simulink model "tb_structure"  (R2026b)
model workspace (MAT data in the model file):
  tbs.t = [0 1000000]
  tbs.uL = [0 0]
  tbs.uR = [0 0]
  tbs.rref = [0 0]
  tbs.pi_on = 0
  tbs.pi_Kp = 0.4
  tbs.pi_Ki = 2
  tbs.pi_lim = 0.4
  tbs.kw = 4.63333333333
  tbs.t_impl = [0 1000000]
  tbs.w_impl = [0 0]
  tbs.nozzleOn = [0; 0; 0; 0; 0; 0; 0; 0]
  tbs.liftDuty = 0
  tbs.envdist.F_ext_B = [0; 0; 0]
  tbs.envdist.M_ext_B = [0; 0; 0]
  tbs.envovr.use_T = 0
  tbs.envovr.T_amb = 318.15
  tbs.envovr.use_G = 0
  tbs.envovr.G_solar = 0
  tbs.envovr.use_soil = 0
  tbs.envovr.soil_id = 2
  tbs.envovr.dock_contact_force = 0
  tbs.decim = 10
undefined symbols (not defined in the file or in its folder): DiscIntNeverNeededParam, Ts
libraries: fl_lib x8, nesl_utility x7
settings Model: Creator=aomar  LastModifiedBy=aomar

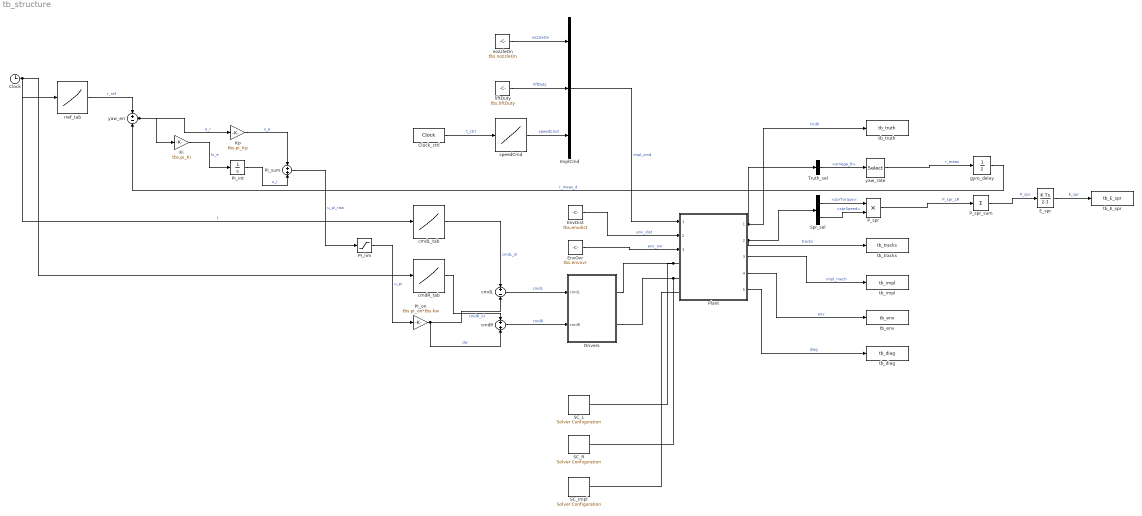
== system tb_structure ==
  Clock : Clock
  Clock_ctrl : DigitalClock  SampleTime=Ts.ctrl
  Drivers : Subsystem  Variant=on  VariantControlMode=label  LabelModeActiveChoice=speed
  E_spr : DiscreteIntegrator  gainval=1  SampleTime=Ts.base  ICPrevOutput=DiscIntNeverNeededParam  ICPrevScaledInput=DiscIntNeverNeededParam
  EnvDist : Constant  Value=tbs.envdist  OutDataTypeStr=Bus: Bus_EnvDisturbance  SampleTime=Ts.base
  EnvOvr : Constant  Value=tbs.envovr  OutDataTypeStr=Bus: Bus_EnvOverride  SampleTime=Ts.env
  ImplCmd : BusCreator  Inputs=3  OutDataTypeStr=Bus: Bus_ImplementCmd  NonVirtualBus=on
  Ki : Gain  Gain=tbs.pi_Ki
  Kp : Gain  Gain=tbs.pi_Kp
  PI_int : Integrator  LimitOutput=on  UpperSaturationLimit=tbs.pi_lim  LowerSaturationLimit=-tbs.pi_lim
  PI_lim : Saturate  UpperLimit=tbs.pi_lim  LowerLimit=-tbs.pi_lim
  PI_on : Gain  Gain=tbs.pi_on*tbs.kw
  PI_sum : Sum
  P_spr : Product  Inputs=**
  P_spr_sum : Sum  Inputs=+
  Plant : Subsystem  ReferencedSubsystem=structure_plant
  SC_Impl : nesl_utility/Solver Configuration  PhysicalDomain=network_engine_domain  SubClassName=solver  LeftPortType=input  RightPortType=generic  Tones=[]  Harmonics=[]  SimulateNoise=off  Profile=off  UseLocalSampling=off  EnableSwitchedLinearOptims=on  FrequencyDomain=off  UseCCode=off  RelTol=0.001  AbsTol=0.001  MinStep=1e-09  ToWorkspace=off  RevertToSquareIcSolve=off  NumHomotopyIterations=100  PhasorMode=off  PhasorModeNumHarmonics=1  ConsistencySolver=NEWTON_XTOL_AFTER_FTOL  CanonicalOrdering=CANONICAL  OptimizeIntermediates=OPTIMIZED  MulticoreSolverChoice=BACKWARD_EULER  IndexReductionMethod=DerivativeReplacement  DoDC=off  ResidualTolerance=1e-09  ConsistencyTolSource=GLOBAL  ConsistencyAbsTol=0.001  ConsistencyRelTol=0.001  ConsistencyTolFactor=0.001  UseLocalSolver=on  LocalSolverChoice=NE_BACKWARD_EULER_ADVANCER  ResolveIndetEquations=on  FunctionEvalNumThread=1  LocalSolverSampleTime=P.sim.ssc.Ts  DoFixedCost=on  MaxNonlinIter=P.sim.ssc.MaxNonlinIter  MaxModeIter=P.sim.ssc.MaxModeIter  ComputeImpulses=off  ImpulseIterations=2  LinearAlgebra=auto  LinearAlgebraNumThread=0  EquationFormulation=NE_TIME_EF  DelaysMemoryBudget=1024  AutomaticFiltering=on  FilteringTimeConstant=0.001  PartitionStorageMethod=AS_NEEDED  PartitionMemoryBudget=1024  PartitionMethod=BALANCED  MultibodyUseLocalSolver=off  MultibodyLocalSolverChoice=ODE1  MultibodyLocalSolverSampleTime=0.001
  SC_L : nesl_utility/Solver Configuration  PhysicalDomain=network_engine_domain  SubClassName=solver  LeftPortType=input  RightPortType=generic  Tones=[]  Harmonics=[]  SimulateNoise=off  Profile=off  UseLocalSampling=off  EnableSwitchedLinearOptims=on  FrequencyDomain=off  UseCCode=off  RelTol=0.001  AbsTol=0.001  MinStep=1e-09  ToWorkspace=off  RevertToSquareIcSolve=off  NumHomotopyIterations=100  PhasorMode=off  PhasorModeNumHarmonics=1  ConsistencySolver=NEWTON_XTOL_AFTER_FTOL  CanonicalOrdering=CANONICAL  OptimizeIntermediates=OPTIMIZED  MulticoreSolverChoice=BACKWARD_EULER  IndexReductionMethod=DerivativeReplacement  DoDC=off  ResidualTolerance=1e-09  ConsistencyTolSource=GLOBAL  ConsistencyAbsTol=0.001  ConsistencyRelTol=0.001  ConsistencyTolFactor=0.001  UseLocalSolver=on  LocalSolverChoice=NE_BACKWARD_EULER_ADVANCER  ResolveIndetEquations=on  FunctionEvalNumThread=1  LocalSolverSampleTime=P.sim.ssc.Ts  DoFixedCost=on  MaxNonlinIter=P.sim.ssc.MaxNonlinIter  MaxModeIter=P.sim.ssc.MaxModeIter  ComputeImpulses=off  ImpulseIterations=2  LinearAlgebra=auto  LinearAlgebraNumThread=0  EquationFormulation=NE_TIME_EF  DelaysMemoryBudget=1024  AutomaticFiltering=on  FilteringTimeConstant=0.001  PartitionStorageMethod=AS_NEEDED  PartitionMemoryBudget=1024  PartitionMethod=BALANCED  MultibodyUseLocalSolver=off  MultibodyLocalSolverChoice=ODE1  MultibodyLocalSolverSampleTime=0.001
  SC_R : nesl_utility/Solver Configuration  PhysicalDomain=network_engine_domain  SubClassName=solver  LeftPortType=input  RightPortType=generic  Tones=[]  Harmonics=[]  SimulateNoise=off  Profile=off  UseLocalSampling=off  EnableSwitchedLinearOptims=on  FrequencyDomain=off  UseCCode=off  RelTol=0.001  AbsTol=0.001  MinStep=1e-09  ToWorkspace=off  RevertToSquareIcSolve=off  NumHomotopyIterations=100  PhasorMode=off  PhasorModeNumHarmonics=1  ConsistencySolver=NEWTON_XTOL_AFTER_FTOL  CanonicalOrdering=CANONICAL  OptimizeIntermediates=OPTIMIZED  MulticoreSolverChoice=BACKWARD_EULER  IndexReductionMethod=DerivativeReplacement  DoDC=off  ResidualTolerance=1e-09  ConsistencyTolSource=GLOBAL  ConsistencyAbsTol=0.001  ConsistencyRelTol=0.001  ConsistencyTolFactor=0.001  UseLocalSolver=on  LocalSolverChoice=NE_BACKWARD_EULER_ADVANCER  ResolveIndetEquations=on  FunctionEvalNumThread=1  LocalSolverSampleTime=P.sim.ssc.Ts  DoFixedCost=on  MaxNonlinIter=P.sim.ssc.MaxNonlinIter  MaxModeIter=P.sim.ssc.MaxModeIter  ComputeImpulses=off  ImpulseIterations=2  LinearAlgebra=auto  LinearAlgebraNumThread=0  EquationFormulation=NE_TIME_EF  DelaysMemoryBudget=1024  AutomaticFiltering=on  FilteringTimeConstant=0.001  PartitionStorageMethod=AS_NEEDED  PartitionMemoryBudget=1024  PartitionMethod=BALANCED  MultibodyUseLocalSolver=off  MultibodyLocalSolverChoice=ODE1  MultibodyLocalSolverSampleTime=0.001
  Spr_sel : BusSelector  OutputSignals=sprTorque,sprSpeed
  Truth_sel : BusSelector  OutputSignals=omega_B
  cmdL : Sum  Inputs=+-
  cmdL_tab : Lookup_n-D  NumberOfTableDimensions=1  BreakpointsForDimension1=tbs.t  Table=tbs.uL  ExtrapMethod=Clip  InternalRulePriority=Speed  RndMeth=Simplest
  cmdR : Sum
  cmdR_tab : Lookup_n-D  NumberOfTableDimensions=1  BreakpointsForDimension1=tbs.t  Table=tbs.uR  ExtrapMethod=Clip  InternalRulePriority=Speed  RndMeth=Simplest
  gyro_delay : UnitDelay  SampleTime=Ts.base
  liftDuty : Constant  Value=tbs.liftDuty  SampleTime=Ts.ctrl
  nozzleOn : Constant  Value=tbs.nozzleOn  OutDataTypeStr=boolean  SampleTime=Ts.ctrl
  rref_tab : Lookup_n-D  NumberOfTableDimensions=1  BreakpointsForDimension1=tbs.t  Table=tbs.rref  ExtrapMethod=Clip  InternalRulePriority=Speed  RndMeth=Simplest
  speedCmd : Lookup_n-D  NumberOfTableDimensions=1  BreakpointsForDimension1=tbs.t_impl  Table=tbs.w_impl  ExtrapMethod=Clip  InternalRulePriority=Speed  RndMeth=Simplest
  tb_E_spr : ToWorkspace  VariableName=tb_E_spr  SaveFormat=Timeseries  SampleTime=-1
      settings: Decimation=tbs.decim
  tb_diag : ToWorkspace  VariableName=tb_diag  SaveFormat=Timeseries  SampleTime=-1
      settings: Decimation=tbs.decim
  tb_env : ToWorkspace  VariableName=tb_env  SaveFormat=Timeseries  SampleTime=-1
      settings: Decimation=tbs.decim
  tb_impl : ToWorkspace  VariableName=tb_impl  SaveFormat=Timeseries  SampleTime=-1
      settings: Decimation=tbs.decim
  tb_tracks : ToWorkspace  VariableName=tb_tracks  SaveFormat=Timeseries  SampleTime=-1
      settings: Decimation=tbs.decim
  tb_truth : ToWorkspace  VariableName=tb_truth  SaveFormat=Timeseries  SampleTime=-1
      settings: Decimation=tbs.decim
  yaw_err : Sum  Inputs=+-
  yaw_rate : Selector  InputPortWidth=3  IndexOptions=Index vector (dialog)  Indices=3  OutputSizes=1
  wires:
  Clock/1 -> cmdR_tab/1, cmdL_tab/1, rref_tab/1  "t"
  rref_tab/1 -> yaw_err/1  "r_ref"
  yaw_err/1 -> Ki/1, Kp/1  "e_r"
  Ki/1 -> PI_int/1  "ki_e"
  Kp/1 -> PI_sum/1  "u_p"
  PI_int/1 -> PI_sum/2  "u_i"
  PI_sum/1 -> PI_lim/1  "u_pi_raw"
  PI_lim/1 -> PI_on/1  "u_pi"
  PI_on/1 -> cmdL/2, cmdR/2  "dw"
  Clock_ctrl/1 -> speedCmd/1  "t_ctrl"
  cmdL_tab/1 -> cmdL/1  "cmdL_ol"
  cmdR_tab/1 -> cmdR/1  "cmdR_ol"
  cmdL/1 -> Drivers/1(cmdL)  "cmdL"
  cmdR/1 -> Drivers/2(cmdR)  "cmdR"
  nozzleOn/1 -> ImplCmd/1  "nozzleOn"
  liftDuty/1 -> ImplCmd/2  "liftDuty"
  speedCmd/1 -> ImplCmd/3  "speedCmd"
  ImplCmd/1 -> Plant/1  "impl_cmd"
  EnvDist/1 -> Plant/2  "env_dist"
  EnvOvr/1 -> Plant/3  "env_ovr"
  Plant/1 -> tb_truth/1, Truth_sel/1  "truth"
  Plant/2 -> Spr_sel/1, tb_tracks/1  "tracks"
  Plant/3 -> tb_impl/1  "impl_mech"
  Plant/4 -> tb_env/1  "env"
  Plant/5 -> tb_diag/1  "diag"
  Truth_sel/1 -> yaw_rate/1  "<omega_B>"
  Spr_sel/1 -> P_spr/1  "<sprTorque>"
  Spr_sel/2 -> P_spr/2  "<sprSpeed>"
  P_spr/1 -> P_spr_sum/1  "P_spr_LR"
  yaw_rate/1 -> gyro_delay/1  "r_meas"
  P_spr_sum/1 -> E_spr/1  "P_spr"
  gyro_delay/1 -> yaw_err/2  "r_meas_d"
  E_spr/1 -> tb_E_spr/1  "E_spr"
  connections:
  Plant/LConn3 -- SC_Impl/RConn1
  Plant/LConn1 -- Drivers/RConn1 -- SC_L/RConn1
  Plant/LConn2 -- Drivers/RConn2 -- SC_R/RConn1

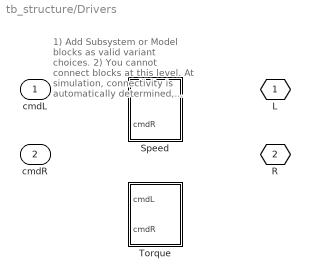
== system tb_structure/Drivers ==
  note: 1) Add Subsystem or Model blocks as valid variant choices.
      | 2) You cannot connect blocks at this level. At simulation, connectivity is automatically
      | determined, based on the active variant and port name matching.
  cmdL : Inport
  cmdR : Inport  Port=2
  Speed : Subsystem  VariantControl=speed
  Torque : Subsystem  VariantControl=torque
  L : PMIOPort  Side=Right  ConnectionType=Connection: foundation.mechanical.rotational.rotational
  R : PMIOPort  Port=2  Side=Right  ConnectionType=Connection: foundation.mechanical.rotational.rotational

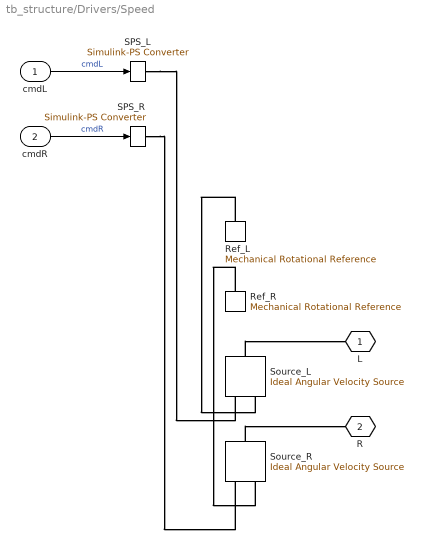
== system tb_structure/Drivers/Speed ==
  cmdL : Inport
  cmdR : Inport  Port=2
  Ref_L : fl_lib/Mechanical/Rotational Elements/Mechanical Rotational Reference
  Ref_R : fl_lib/Mechanical/Rotational Elements/Mechanical Rotational Reference
  SPS_L : nesl_utility/Simulink-PS Converter  PhysicalDomain=network_engine_domain  SubClassName=ps_input  LeftPortType=input  RightPortType=output  PseudoPeriodic=off  Frequencies=[]  NoiseDistribution=none  NoiseParameters=[]  Unit=rad/s  AffineConversion=off  FilteringAndDerivatives=filter  SimscapeFilterOrder=1  InputFilterTimeConstant=P.sim.ssc.tau_filt  UdotUserProvided=0
  SPS_R : nesl_utility/Simulink-PS Converter  PhysicalDomain=network_engine_domain  SubClassName=ps_input  LeftPortType=input  RightPortType=output  PseudoPeriodic=off  Frequencies=[]  NoiseDistribution=none  NoiseParameters=[]  Unit=rad/s  AffineConversion=off  FilteringAndDerivatives=filter  SimscapeFilterOrder=1  InputFilterTimeConstant=P.sim.ssc.tau_filt  UdotUserProvided=0
  Source_L : fl_lib/Mechanical/Mechanical Sources/Ideal Angular Velocity Source
  Source_R : fl_lib/Mechanical/Mechanical Sources/Ideal Angular Velocity Source
  L : PMIOPort  Side=Right  ConnectionType=Connection: foundation.mechanical.rotational.rotational
  R : PMIOPort  Port=2  Side=Right  ConnectionType=Connection: foundation.mechanical.rotational.rotational
  wires:
  cmdL/1 -> SPS_L/1  "cmdL"
  cmdR/1 -> SPS_R/1  "cmdR"
  connections:
  Source_L/LConn1 -- L/RConn1
  Source_R/LConn1 -- R/RConn1
  Ref_L/LConn1 -- Source_L/RConn2
  Ref_R/LConn1 -- Source_R/RConn2
  SPS_L/RConn1 -- Source_L/RConn1
  SPS_R/RConn1 -- Source_R/RConn1

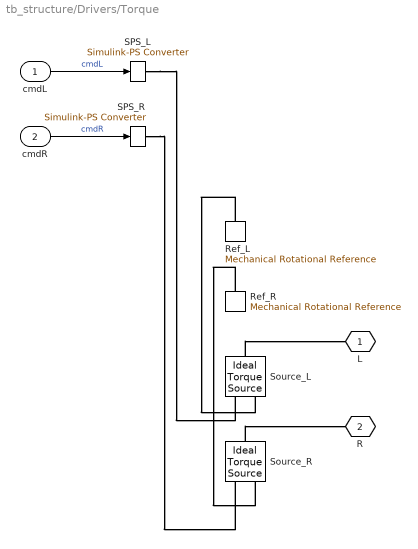
== system tb_structure/Drivers/Torque ==
  cmdL : Inport
  cmdR : Inport  Port=2
  Ref_L : fl_lib/Mechanical/Rotational Elements/Mechanical Rotational Reference
  Ref_R : fl_lib/Mechanical/Rotational Elements/Mechanical Rotational Reference
  SPS_L : nesl_utility/Simulink-PS Converter  PhysicalDomain=network_engine_domain  SubClassName=ps_input  LeftPortType=input  RightPortType=output  PseudoPeriodic=off  Frequencies=[]  NoiseDistribution=none  NoiseParameters=[]  Unit=N*m  AffineConversion=off  FilteringAndDerivatives=zero  SimscapeFilterOrder=1  InputFilterTimeConstant=0.001  UdotUserProvided=0
  SPS_R : nesl_utility/Simulink-PS Converter  PhysicalDomain=network_engine_domain  SubClassName=ps_input  LeftPortType=input  RightPortType=output  PseudoPeriodic=off  Frequencies=[]  NoiseDistribution=none  NoiseParameters=[]  Unit=N*m  AffineConversion=off  FilteringAndDerivatives=zero  SimscapeFilterOrder=1  InputFilterTimeConstant=0.001  UdotUserProvided=0
  Source_L : fl_lib/Mechanical/Mechanical Sources/Ideal Torque Source
  Source_R : fl_lib/Mechanical/Mechanical Sources/Ideal Torque Source
  L : PMIOPort  Side=Right  ConnectionType=Connection: foundation.mechanical.rotational.rotational
  R : PMIOPort  Port=2  Side=Right  ConnectionType=Connection: foundation.mechanical.rotational.rotational
  wires:
  cmdL/1 -> SPS_L/1  "cmdL"
  cmdR/1 -> SPS_R/1  "cmdR"
  connections:
  Source_L/LConn1 -- L/RConn1
  Source_R/LConn1 -- R/RConn1
  Ref_L/LConn1 -- Source_L/RConn2
  Ref_R/LConn1 -- Source_R/RConn2
  SPS_L/RConn1 -- Source_L/RConn1
  SPS_R/RConn1 -- Source_R/RConn1
